simulink model "MATE_HDLsolver_my4thCircuit"  (R2024b)
settings: Solver=FixedStepDiscrete  StartTime=0.0  StopTime=0.05  FixedStep=Ts  MaxStep=100e-6  RelTol=1e-4
PostLoadFcn:
  | Ts=1e-6; nb_sw=3; nb_lc=2;nb_r=1;nb_src=1; nb_out=3; rL=1.2;rC=100;L=1e-3; C=1e-5; Cx=C;LpejoSw=1e-6;h=Ts; MAX_INPUTS=16;
  | MAX_OUTPUTS=16;
  | MAX_SWITCHES=8;
  | MAX_INPUTS=16;
InitFcn:
  | Ts=1e-6; nb_sw=3; nb_lc=2;nb_r=1;nb_src=1; nb_out=3; rL=1.2;rC=100;L=1e-3; C=1e-5; Cx=C;LpejoSw=1e-6;h=Ts; MAX_INPUTS=16;
  | MAX_OUTPUTS=16;
  | MAX_SWITCHES=8;
  | MAX_INPUTS=16;
undefined symbols (not defined in the file or in its folder): MATE_SOC
libraries: fl_lib x35, nesl_utility x13, simetranss x6, ee_lib x4, simulink x3, hdlsllib x3, eeGeneralControl x1
Description:
  | Copyright 2008-2010 The MathWorks, Inc.
settings Model: ARTEMISmethode_block_infos=$$__separator__$$  ModifiedByFormat=Kyle  Creator=Kyle Diller  LastModifiedBy=Kyle
settings SolverCC: AlgebraicLoopSolver=TrustRegion
settings DataIOCC: SaveFormat=Array  SignalLoggingSaveFormat=ModelDataLogs  ReturnWorkspaceOutputs=off  SignalLoggingName=sigsOut
settings OptimizationCC: BlockReduction=off  ConditionallyExecuteInputs=off  OptimizeBlockIOStorage=off  BufferReuse=off  GlobalBufferReuse=off  ExpressionFolding=off  ExpressionDepthLimit=2147483647  LocalBlockOutputs=off  InitFltsAndDblsToZero=on  LifeSpan=inf
settings DebuggingCC: SaveWithParameterizedLinksMsg=none  UnderspecifiedInitializationDetection=Classic  MergeDetectMultiDrivingBlocksExec=none  CheckExecutionContextPreStartOutputMsg=on  SignalResolutionControl=TryResolveAllWithWarning  MultiTaskDSMMsg=warning  MultiTaskCondExecSysMsg=none  SingleTaskRateTransMsg=error  SigSpecEnsureSampleTimeMsg=none  FcnCallInpInsideContextMsg=warning  UnconnectedInputMsg=warning  UnconnectedOutputMsg=warning  UnconnectedLineMsg=warning  AllowSymbolicDim=off  StateNameClashWarn=warning  SFUnexpectedBacktrackingDiag=warning  SFNoUnconditionalDefaultTransitionDiag=warning  SFExecutionAtInitializationDiag=none  ArithmeticOperatorsInVariantConditions=warning
settings HardwareCC: ProdBitPerPointer=32  ProdBitPerSizeT=32  ProdBitPerPtrDiffT=32  ProdLargestAtomicFloat=None  ProdIntDivRoundTo=Undefined  ProdEndianess=Unspecified  ProdWordSize=32  ProdHWDeviceType=Specified  TargetUnknown=on
settings ModelReferenceCC: EnableRefExpFcnMdlSchedulingChecks=on  PropagateSignalLabelsOutOfModel=off
settings SFSimCC: SimUseLocalCustomCode=off  CustomCodeUndefinedFunction=UseInterfaceOnly
settings RTWCC: RTWUseLocalCustomCode=off  GPUComputeCapability=3.5
settings CodeAppCC: StateflowObjectComments=on
settings GRTTargetCC: TargetFcnLib=ansi_tfl_tmw.mat  TargetLangStandard=C89/C90 (ANSI)  CombineOutputUpdateFcns=off  GRTInterface=on
settings ConfigComp: CovMetricSettings=dw  CovSaveCumulativeToWorkspaceVar=on  CovSaveSingleToWorkspaceVar=on  CovExternalEMLEnable=off
settings SimscapeCC: SimscapeNormalizeSystem=off

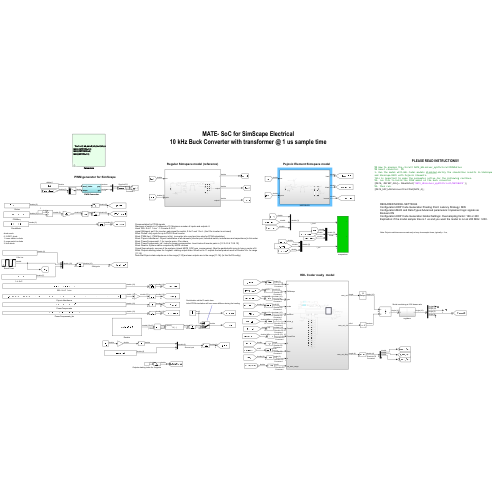
[thumbnail: Simulink's stored preview of the top-level diagram]
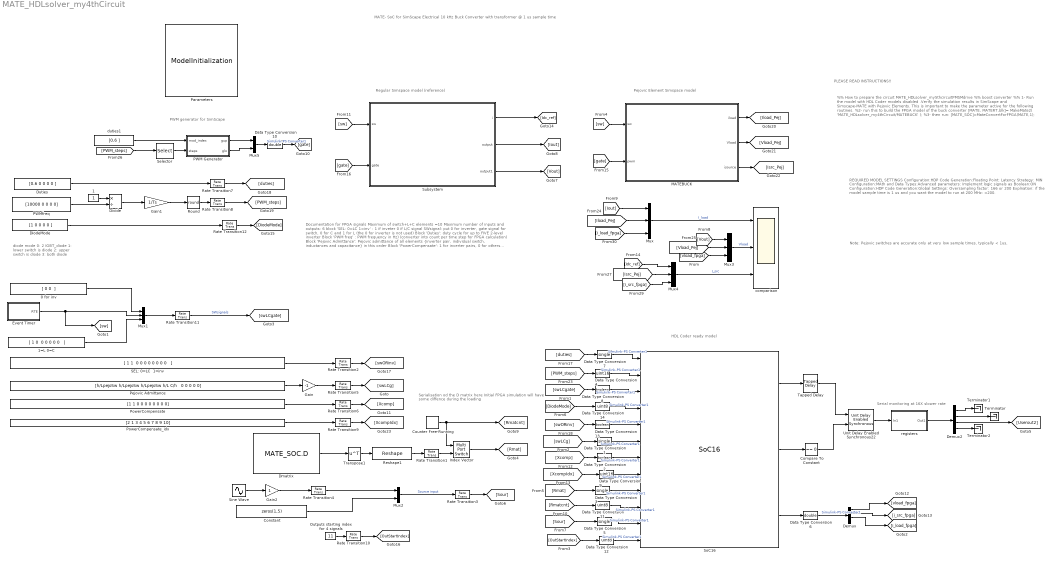
== system MATE_HDLsolver_my4thCircuit ==
  note: Documentation for FPGA signals
      | Maximum of switch+L+C elements =10 Maximum number of inputs and outputs: 6
      | block 'SEL: 0=LC 1=inv' : 1 if inveter 0 if L/C
      | signal SWsignal: put 0 for inverter, gate signal for switch, 0 for C and 1 for L (the 0 for inverter is not used)
      | Block 'Duties': duty cycle for up to FIVE 2-level inverter
      | Block 'PWM freq' : PWM frequency in Hz) (converter into count per time step for FPGA calculation)
      | Block 'Pejovic Admittance': Pejovic admittance of all elements {inverter pair, individual switch, inductances and capacitance} in this order
      | Block 'PowerCompensate': 1 for inverter pairs, 0 for others
      | Block 'PowerCompensate_idx': index for power compensation. Invert index of inverter pairs in [1 2 3 4 5 6 7 8 9 10]
      | Block Dmatrix: System matrix computed by MATE routines
      | Signal SourceInputs: sources of the systems (check MATE_SOC.new_sourcenames). Must be padded with zeros to have a vector of 6
      | Block 'Outputs starting index for 4 signals': starting output index. When set to 11 outputs the last product result of Dmatrix*Vin. for range [11:14]
      | Note that Pejovic state outputs are in the range [1:10] and user outputs are in the range [11:16]. (In this SoCS config)
  note: Serial monitoring at 16X slower rate
  note: Serialisation od the D matrix here
      | Initial FPGA simulation will have some diffence during the loading
  note: Regular Simspace model (reference)
  note: Note: Pejovic switches are accurate only at very low sample times, typically < 1us,
  note: Pejovic Element Simspace model
  note: PLEASE READ INSTRUCTIONS!!
  note: %% How to prepare the circuit MATE_HDLsolver_my5thcircuitPMSMdrive
      | %% boost converter %%
      | 1- Run the model with HDL Coder models disabled .Verify the simulation results in SimScape and Simscape-MATE with Pejovic Elements.
      | This is important to make the parameter active for the following routines.
      | %2- run this to build the FPGA model of the buck converter
      | [MATE, MATERT,blk]= MakeMate2( 'MATE_HDLsolver_my4thCircuit/MATEBUCK' );
      | %3- then run:
      | [MATE_SOC]=MateConvertForFPGA(MATE,1);
  note: HDL Coder ready model
  note: MATE- SoC for SimScape Electrical
      | 10 kHz Buck Converter with transformer @ 1 us sample time
  note: PWM generator for SimScape
  note: diode mode
      | 0: 2 IGBT_diode
      | 1: lower switch is diode
      | 2: upper switch is diode
      | 3: both diode
  note: REQUIRED MODEL SETTINGS
      | Configuration:HDP Code Generation:Floating Point: Latency Strategy: MIN
      | Configuration:MAth and Data Types:Advanced parameters: Implement logic signals as Boolean:ON
      | Configuration:HDP Code Generation:Global Settings: Oversampling factor: 166 or 200
      | Explnation: if the model sample time is 1 us and you want the model to run at 200 MHz: =200.
  " Event Timer" : Subsystem  Tag=RTEcontrol_s38shd7k88  LoadFcn=|  mask(Timer){is=0 (off), t=[0.01 0.02 0.03 0.04 ], Tmax=0.07, Ts=Ts}
      | xx=get_param(gcb,'linkstatus');      
      | if isequal(xx,'inactive')            
      | set_param(gcb,'linkstatus','restore')
      | end
      mask prompts: is "Initial state"; t "Transition times (s):"; Tmax "Repeat period (s)"; Ts "Sample time (s)"
      mask help: This block generates a Simulink control signal changing at specified transition times.
      mask init:
      | iss=get_param(gcb,'is');
      | if isequal(iss,'0 (off)')
      |     sw(1)=0;
      |     sw(2)=0;
      | else
      |     sw(1)=1;
      |     sw(2)=1;
      | end
      | st(1)=0;
      | st(2)=t(1);
      | 
      | if t(1)==0,
      |    h=errordlg(' The first time specified must be greater than 0 ' , 'Parameter error');
      | end
      | 
      | i=3;
      | tog=0;
      | ptr=2;
      | while length(sw)<=2*length(t)
      |     if tog==0
      |         st=[st st(end)+Ts];
      |         sw=[sw 1-sw(end)];
      |         tog=1;
      |     else
      |         st=[st t(ptr)];
      |         sw=[sw sw(end)];
      |         ptr=ptr+1;
      |         tog=0;
      |     end
      | 
      | end
      |  %st=[st Tmax-Ts Tmax+Ts]
      | % sw=[sw sw(end) sw(1)]
      mask TypeOptions is: 0 (off) | 1 (on)
      mask Display:
      | %plot(0,0,100,100,[70,40,40,20,20,13],[30,30,70,70,30,30]);
      | plot( st(1:end-1), sw(1:end-1) );
  0 for inv : Constant  Value="[ 0 0  ]"
  1 : Constant
  1=L 0=C : Constant  Value="[ 1 0  0 0 0 0 0   ]"
  Compare To Constant : hdlsllib/Logic and Bit Operations/Compare To Constant  relop===  const=0  OutDataTypeStr=boolean
  Constant : Constant  Value=zeros(1,5)
  Counter Free-Running : hdlsllib/Sources/Counter Free-Running  NumBits=8  tsamp=-1
  Data Type Conversion{1,3,5,7} (4 alike) : DataTypeConversion  OutDataTypeStr=single  RndMeth=Nearest  SaturateOnIntegerOverflow=off
  Data Type Conversion10 : DataTypeConversion  OutDataTypeStr=double  RndMeth=Nearest  SaturateOnIntegerOverflow=off
  Data Type Conversion11 : DataTypeConversion  OutDataTypeStr=uint8  RndMeth=Nearest  SaturateOnIntegerOverflow=off
  Data Type Conversion12 : DataTypeConversion  OutDataTypeStr=uint8  RndMeth=Nearest  SaturateOnIntegerOverflow=off
  Data Type Conversion13 : DataTypeConversion  OutDataTypeStr=boolean  RndMeth=Nearest  SaturateOnIntegerOverflow=off
  Data Type Conversion14 : DataTypeConversion  OutDataTypeStr=uint8  RndMeth=Nearest  SaturateOnIntegerOverflow=off
  Data Type Conversion2 : DataTypeConversion  OutDataTypeStr=boolean  RndMeth=Nearest  SaturateOnIntegerOverflow=off
  Data Type Conversion4 : DataTypeConversion  OutDataTypeStr=uint16  RndMeth=Nearest  SaturateOnIntegerOverflow=off
  Data Type Conversion6 : DataTypeConversion  OutDataTypeStr=double  RndMeth=Nearest  SaturateOnIntegerOverflow=off
  Data Type Conversion8 : DataTypeConversion  OutDataTypeStr=boolean  RndMeth=Nearest  SaturateOnIntegerOverflow=off
  Data Type Conversion9 : DataTypeConversion  OutDataTypeStr=uint16  RndMeth=Nearest  SaturateOnIntegerOverflow=off
  Demux : Demux
  Demux2 : Demux  Outputs=[nb_sw nb_lc nb_out MAX_OUTPUTS-nb_out-nb_sw-nb_lc]
  DiodeMode : Constant  Value=[1 0 0 0 0 ]
  Divide : Product  Inputs=*/
  Dmatrix : Constant  Value=MATE_SOC.D
  Duties : Constant  Value=[0.6 0 0 0 0 ]
  Gain : Gain  Gain=-1
  Gain1 : Gain  Gain=1/Ts
  Gain2 : Gain
  Index Vector : MultiPortSwitch  DataPortOrder=Zero-based contiguous  Inputs=1  zeroidx=on  SaturateOnIntegerOverflow=off  InputSameDT=off
  MATEBUCK : Subsystem
  Mux{,1,3..4} (4 alike) : Mux  Inputs=3
  Mux2 : Mux  Inputs=2
  Mux5 : Mux  Inputs=2
  Outputs starting index for 4 signals : Constant  Value=11
  PWM Generator : Subsystem  Tag=RTEcontrol_s38shd7k88
  PWMfreq : Constant  Value=[10000 0 0 0 0]
  Parameters : simetranss/Usefulls/ModelInitialization  InitFcnX=|  prel=off  posl=on  inif=on  strf=off
      | Ts=1e-6; nb_sw=3; nb_lc=2;nb_r=1;nb_src=1; nb_out=3; rL=1.2;rC=100;L=1e-3; C=1e-5; Cx=C;LpejoSw=1e-6;h=Ts; MAX_INPUTS=16;
      | MAX_OUTPUTS=16;
      | MAX_SWITCHES=8;
      | MAX_INPUTS=16;
  Pejovic Admittance : Constant  Value="[h/LpejoSw h/LpejoSw h/LpejoSw h/L C/h   0 0 0 0 0]"
  PowerCompensate : Constant  Value=[1 1 0 0 0 0 0 0 0 0]
  PowerCompensate_idx : Constant  Value=[2 1 3 4 5 6 7 8 9 10]
  Rate Transition{1..12} (12 alike) : RateTransition  OutPortSampleTime=1e-06
  Reshape1 : Reshape
  Round : Rounding  Operator=round
  SEL: 0=LC  1=inv : Constant  Value="[ 1 1  0 0 0 0 0 0 0 0   ]"
  Selector : Selector  InputPortWidth=5  IndexOptions=Index vector (dialog)  Indices=1  OutputSizes=1
  Sine Wave : Sin  Amplitude=0  Bias=100  Frequency=0  SampleTime=0
  SoC16 : simetranss/SoC/SoC16  SystemSampleTime=-1  VariantActivationTime=update diagram  AllowFlexibleInterface=on  Latency=0  AutoFrameSizeCalculation=off
  Subsystem : Subsystem
  Tapped Delay : simulink/Discrete/Tapped Delay  vinit=0.0  samptime=-1  NumDelays=16  DelayOrder=Oldest  includeCurrent=off
      settings: LibrarySourceBlock=hdlsllib/Discrete/Tapped Delay
  Terminator : Terminator
  Terminator1 : Terminator
  Terminator2 : Terminator
  Transpose1 : Math  Operator=transpose
  Unit Delay Enabled Synchronous22 : hdlsllib/Discrete/Unit Delay Enabled Synchronous  InitialCondition=0.0  SampleTime=-1
  comparison : Scope  NumInputPorts=3
  duties1 : Constant  Value=[0.6 ]
  registers : Subsystem
  wires:
  Mux/1 -> comparison/1  "I_load"
  Dmatrix/1 -> Transpose1/1
  Sine Wave/1 -> Gain2/1
  Mux3/1 -> comparison/2  "Vload"
  [Vout] -> Mux3/1
  [sw] -> MATEBUCK/1(sw)
  Mux1/1 -> Rate Transition11/1
  Pejovic Admittance/1 -> Gain/1
  Rate Transition5/1 -> [swLCg]
  Gain2/1 -> Rate Transition4/1
  Rate Transition6/1 -> [Xcomp]
  PowerCompensate/1 -> Rate Transition6/1
  [vload_fpga] -> Mux3/3
  [gate] -> MATEBUCK/2(pwm)
  Duties/1 -> Rate Transition7/1
  Rate Transition7/1 -> [duties]
  Mux2/1 -> Rate Transition3/1  "Source input"
  Rate Transition4/1 -> Mux2/1
  Constant/1 -> Mux2/2
  Rate Transition8/1 -> [PWM_steps]
  Divide/1 -> Gain1/1
  Gain1/1 -> Round/1
  Demux2/2 -> Terminator/1
  MATEBUCK/1(iload) -> [Iload_Pej]
  MATEBUCK/2(Vload) -> [Vload_Pej]
  MATEBUCK/3(isource) -> [Isrc_Pej]
  [Iload_Pej] -> Mux/2
  [i_load_fpga] -> Mux/3
  [Vload_Pej] -> Mux3/2
  Mux4/1 -> comparison/3  "I_src"
  [Idc_ref] -> Mux4/1
  [Isrc_Pej] -> Mux4/2
  Demux2/3 -> [Userout2]
  Demux2/1 -> Terminator1/1
  Demux2/4 -> Terminator2/1
  PWMfreq/1 -> Divide/2
  1/1 -> Divide/1
  [i_src_fpga] -> Mux4/3
  PowerCompensate_idx/1 -> Rate Transition9/1
  Rate Transition9/1 -> [XcompIdx]
  Round/1 -> Rate Transition8/1
  duties1/1 -> PWM Generator/1(mod_index)
  [PWM_steps] -> Selector/1
  PWM Generator/2(glo) -> Mux5/2
  PWM Generator/1(gup) -> Mux5/1
  Mux5/1 -> Data Type Conversion10/1
  Data Type Conversion10/1 -> [gate]  "Simulink-PS Converter1"
  [Iout] -> Mux/1
  Transpose1/1 -> Reshape1/1
  Reshape1/1 -> Rate Transition1/1
  Rate Transition1/1 -> Index Vector/2
  Counter Free-Running/1 -> Index Vector/1, [Rmatcnt]
  Index Vector/1 -> [Rmat]
  [Rmatcnt] -> Data Type Conversion11/1
  [swLCg] -> Data Type Conversion1/1
  [XcompIdx] -> Data Type Conversion9/1
  [swLCgate] -> Data Type Conversion8/1
  [Xcomp] -> Data Type Conversion2/1
  [Sour] -> Data Type Conversion5/1
  [Rmat] -> Data Type Conversion3/1
  [duties] -> Data Type Conversion7/1
  Data Type Conversion8/1 -> SoC16/3  "Simulink-PS Converter1"
  Data Type Conversion2/1 -> SoC16/7  "Simulink-PS Converter1"
  Data Type Conversion5/1 -> SoC16/11  "Simulink-PS Converter1"
  Data Type Conversion3/1 -> SoC16/9  "Simulink-PS Converter1"
  [PWM_steps] -> Data Type Conversion4/1
  Data Type Conversion1/1 -> SoC16/6  "Simulink-PS Converter1"
  Data Type Conversion9/1 -> SoC16/8  "Simulink-PS Converter1"
  Data Type Conversion4/1 -> SoC16/2  "Simulink-PS Converter1"
  Data Type Conversion11/1 -> SoC16/10  "Simulink-PS Converter1"
  Data Type Conversion7/1 -> SoC16/1  "Simulink-PS Converter1"
  [gate] -> Subsystem/2(gate)
  Subsystem/1(i) -> [Idc_ref]
  Subsystem/2(output) -> [Iout]
  Subsystem/3(output1) -> [Vout]
  Tapped Delay/1 -> Unit Delay Enabled Synchronous22/1
  SoC16/2 -> Compare To Constant/1
  SoC16/1 -> Tapped Delay/1
  Compare To Constant/1 -> Unit Delay Enabled Synchronous22/2
  Unit Delay Enabled Synchronous22/1 -> registers/1(In1)
  registers/1(Out1) -> Demux2/1
  [OutStartIndex] -> Data Type Conversion12/1
  Data Type Conversion12/1 -> SoC16/12  "Simulink-PS Converter1"
  Rate Transition10/1 -> [OutStartIndex]
  Outputs starting index for 4 signals/1 -> Rate Transition10/1
  [sw] -> Subsystem/1(sw)
  0 for inv/1 -> Mux1/1
  " Event Timer"/1(RTE) -> Mux1/2, [sw]
  Rate Transition11/1 -> [swLCgate]  "SWsignals"
  1=L 0=C/1 -> Mux1/3
  Rate Transition2/1 -> [swORinv]
  SEL: 0=LC  1=inv/1 -> Rate Transition2/1
  [swORinv] -> Data Type Conversion13/1
  Data Type Conversion13/1 -> SoC16/5  "Simulink-PS Converter1"
  Rate Transition3/1 -> [Sour]
  Selector/1 -> PWM Generator/2(steps)
  Gain/1 -> Rate Transition5/1
  Demux/3 -> [i_load_fpga]
  Data Type Conversion6/1 -> Demux/1  "Simulink-PS Converter1"
  Demux/1 -> [vload_fpga]
  Demux/2 -> [i_src_fpga]
  SoC16/3 -> Data Type Conversion6/1
  Rate Transition12/1 -> [DiodeMode]
  DiodeMode/1 -> Rate Transition12/1
  [DiodeMode] -> Data Type Conversion14/1
  Data Type Conversion14/1 -> SoC16/4  "Simulink-PS Converter1"

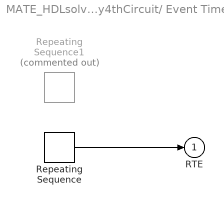
== system MATE_HDLsolver_my4thCircuit/ Event Timer ==
  Repeating Sequence : simulink/Sources/Repeating Sequence  rep_seq_t=st  rep_seq_y=sw
  Repeating Sequence1 : simulink/Sources/Repeating Sequence  Commented=on  rep_seq_t="[0    0.2000    0.2001    0.4000    0.4001    0.6000    2.0000]"  rep_seq_y=|
      | [     1     1     0     0     1     1     1
      | ]
  RTE : Outport  VectorParamsAs1DForOutWhenUnconnected=off
  wires:
  Repeating Sequence/1 -> RTE/1

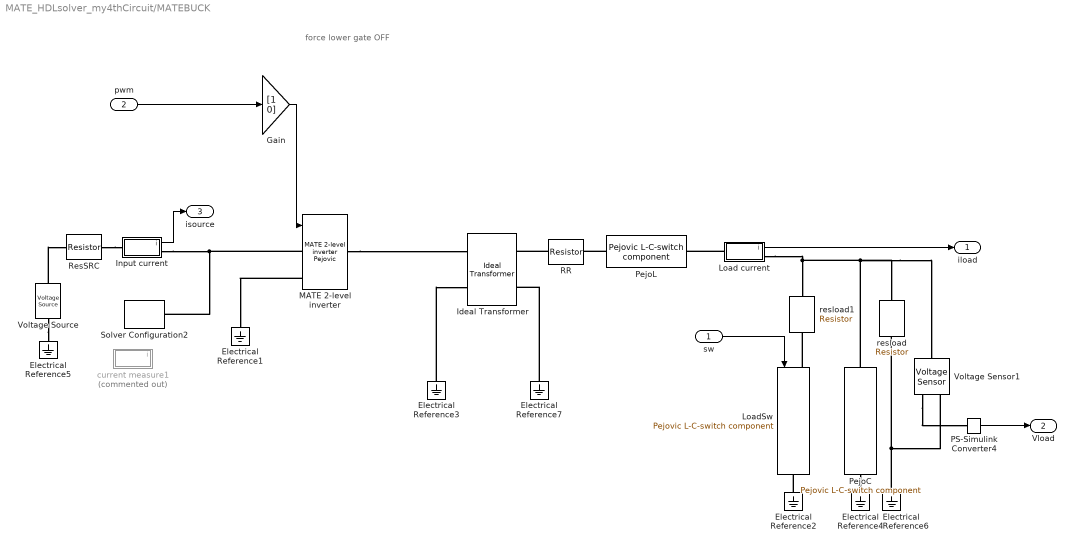
== system MATE_HDLsolver_my4thCircuit/MATEBUCK ==
  note: force lower gate OFF
  sw : Inport
  pwm : Inport  Port=2
  Electrical Reference{1..7} (7 alike) : fl_lib/Electrical/Electrical Elements/Electrical Reference
  Gain : Gain  Gain=[1 0]
  Ideal Transformer : fl_lib/Electrical/Electrical Elements/Ideal Transformer  n=2  i1_specify=off  i1_priority=None  i1=0 A  i1_nominal_specify=off  i1_nominal_value=1  i1_nominal_unit=A  v1_specify=off  v1_priority=None  v1=0 V  v1_nominal_specify=off  v1_nominal_value=1  v1_nominal_unit=V  i2_specify=off  i2_priority=None  i2=0 A  i2_nominal_specify=off  i2_nominal_value=1  i2_nominal_unit=A  v2_specify=off  v2_priority=None  v2=0 V  v2_nominal_specify=off  v2_nominal_value=1  v2_nominal_unit=V
  Input current : Subsystem
  Load current : Subsystem
  LoadSw : simetranss/FPGA/Pejovic L-C-switch component  typ=Switch  Lon=LpejoSw  L=L  C=Cx  traprule=off  otherSW='coming soon'  Ts=Ts  pcbp=off  showV=off  showI=off
  MATE 2-level inverter : simetranss/FPGA/MATE 2-level inverter Pejovic  Lon=1e-6  Ts=Ts
  PS-Simulink Converter4 : nesl_utility/PS-Simulink Converter  PhysicalDomain=network_engine_domain  SubClassName=ps_output  LeftPortType=input  RightPortType=output  PseudoPeriodic=off  Frequencies=[]  VectorFormat=inherit  Unit=inherit  AffineConversion=off
  PejoC : simetranss/FPGA/Pejovic L-C-switch component  typ=Capacitor  Lon=LpejoSw  L=L  C=Cx  traprule=off  otherSW='coming soon'  Ts=Ts  pcbp=off  showV=off  showI=off
  PejoL : simetranss/FPGA/Pejovic L-C-switch component  typ=Inductor  Lon=LpejoSw  L=L  C=C  traprule=off  otherSW='coming soon'  Ts=Ts  pcbp=off  showV=off  showI=off
  RR : fl_lib/Electrical/Electrical Elements/Resistor  R=rL Ohm  i_specify=off  i_priority=None  i=0 A  i_nominal_specify=off  i_nominal_value=1  i_nominal_unit=A  v_specify=off  v_priority=None  v=0 V  v_nominal_specify=off  v_nominal_value=1  v_nominal_unit=V
  ResSRC : fl_lib/Electrical/Electrical Elements/Resistor  R=0.01 Ohm  i_specify=off  i_priority=None  i=0 A  i_nominal_specify=off  i_nominal_value=1  i_nominal_unit=A  v_specify=off  v_priority=None  v=0 V  v_nominal_specify=off  v_nominal_value=1  v_nominal_unit=V
  Solver Configuration2 : nesl_utility/Solver Configuration  PhysicalDomain=network_engine_domain  SubClassName=solver  LeftPortType=input  RightPortType=generic  Tones=[]  Harmonics=[]  SimulateNoise=off  Profile=off  UseLocalSampling=off  EnableSwitchedLinearOptims=on  FrequencyDomain=off  UseCCode=off  RelTol=0.001  AbsTol=0.001  MinStep=1e-09  ToWorkspace=off  RevertToSquareIcSolve=off  NumHomotopyIterations=100  PhasorMode=off  PhasorModeNumHarmonics=1  ConsistencySolver=NEWTON_XTOL_AFTER_FTOL  IndexReductionMethod=DerivativeReplacement  DoDC=off  ResidualTolerance=1e-09  ConsistencyTolSource=GLOBAL  ConsistencyAbsTol=0.001  ConsistencyRelTol=0.001  ConsistencyTolFactor=0.001  UseLocalSolver=on  LocalSolverChoice=NE_BACKWARD_EULER_ADVANCER  ResolveIndetEquations=on  FunctionEvalNumThread=1  LocalSolverSampleTime=Ts  DoFixedCost=on  MaxNonlinIter=1  MaxModeIter=2  ComputeImpulses=off  ImpulseIterations=2  LinearAlgebra=auto  LinearAlgebraNumThread=0  EquationFormulation=NE_TIME_EF  DelaysMemoryBudget=1024  AutomaticFiltering=on  FilteringTimeConstant=0.001  PartitionStorageMethod=AS_NEEDED  PartitionMemoryBudget=1024  PartitionMethod=ROBUST  MultibodyUseLocalSolver=off  MultibodyLocalSolverChoice=ODE1  MultibodyLocalSolverSampleTime=0.001
  Voltage Sensor1 : fl_lib/Electrical/Electrical Sensors/Voltage Sensor
  Voltage Source : ee_lib/Sources/Voltage Source  dc_voltage=100 V  ac_voltage=0 V  ac_shift=0 rad  ac_frequency=60 Hz  noise_mode=ee.enum.sources.noise.Disabled  PSD=0 V^2/Hz  sample_time=1e-3 s  repeatability=ee.enum.sources.repeatability.NotRepeatable  user_seed=0  auto_seed=198304613  i_specify=off  i_priority=None  i=0 A  i_nominal_specify=off  i_nominal_value=1  i_nominal_unit=A  v_specify=off  v_priority=None  v=0 V  v_nominal_specify=off  v_nominal_value=1  v_nominal_unit=V
  current measure1 : Subsystem  Commented=on
      mask Display: disp('amp')
  resload : fl_lib/Electrical/Electrical Elements/Resistor  R=rC Ohm  i_specify=off  i_priority=None  i=0 A  i_nominal_specify=off  i_nominal_value=1  i_nominal_unit=A  v_specify=off  v_priority=None  v=0 V  v_nominal_specify=off  v_nominal_value=1  v_nominal_unit=V
  resload1 : fl_lib/Electrical/Electrical Elements/Resistor  R=rC Ohm  i_specify=off  i_priority=None  i=0 A  i_nominal_specify=off  i_nominal_value=1  i_nominal_unit=A  v_specify=off  v_priority=None  v=0 V  v_nominal_specify=off  v_nominal_value=1  v_nominal_unit=V
  iload : Outport
  Vload : Outport  Port=2
  isource : Outport  Port=3
  wires:
  PS-Simulink Converter4/1 -> Vload/1
  sw/1 -> LoadSw/1
  Load current/1(i) -> iload/1
  pwm/1 -> Gain/1
  Input current/1(i) -> isource/1
  Gain/1 -> MATE 2-level inverter/1
  connections:
  Load current/LConn1 -- PejoL/RConn1
  Voltage Source/RConn1 -- Electrical Reference5/LConn1
  Voltage Source/LConn1 -- ResSRC/LConn1
  PejoL/LConn1 -- RR/RConn1
  PejoC/RConn1 -- Electrical Reference4/LConn1
  Voltage Sensor1/RConn1 -- PS-Simulink Converter4/LConn1
  Electrical Reference6/LConn1 -- resload/RConn1 -- Voltage Sensor1/RConn2
  Input current/RConn1 -- MATE 2-level inverter/LConn1 -- Solver Configuration2/RConn1
  Voltage Sensor1/LConn1 -- resload/LConn1 -- Load current/RConn1 -- resload1/LConn1 -- PejoC/LConn1
  MATE 2-level inverter/LConn2 -- Electrical Reference1/LConn1
  LoadSw/LConn1 -- resload1/RConn1
  Electrical Reference2/LConn1 -- LoadSw/RConn1
  ResSRC/RConn1 -- Input current/LConn1
  RR/LConn1 -- Ideal Transformer/RConn1
  Electrical Reference3/LConn1 -- Ideal Transformer/LConn2
  Electrical Reference7/LConn1 -- Ideal Transformer/RConn2
  MATE 2-level inverter/RConn1 -- Ideal Transformer/LConn1

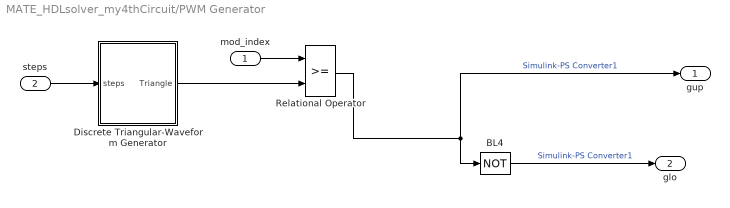
== system MATE_HDLsolver_my4thCircuit/PWM Generator ==
  mod_index : Inport
  steps : Inport  Port=2
  BL4 : Logic  Operator=NOT  Inputs=1
  Discrete Triangular-Waveform Generator : Subsystem
  Relational Operator : RelationalOperator  OutDataTypeStr=boolean
  gup : Outport  VectorParamsAs1DForOutWhenUnconnected=off
  glo : Outport  Port=2  VectorParamsAs1DForOutWhenUnconnected=off
  wires:
  Discrete Triangular-Waveform Generator/1(Triangle) -> Relational Operator/2
  mod_index/1 -> Relational Operator/1
  steps/1 -> Discrete Triangular-Waveform Generator/1(steps)
  Relational Operator/1 -> gup/1, BL4/1  "Simulink-PS Converter1"
  BL4/1 -> glo/1  "Simulink-PS Converter1"

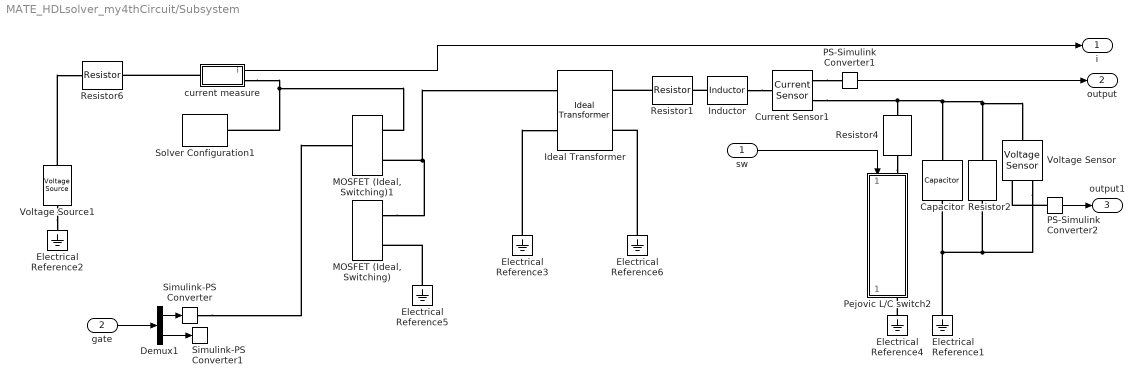
== system MATE_HDLsolver_my4thCircuit/Subsystem ==
  sw : Inport
  gate : Inport  Port=2
  Capacitor : fl_lib/Electrical/Electrical Elements/Capacitor  c=C F  r=0 Ohm  g=0 1/Ohm  i_specify=off  i_priority=None  i=0 A  i_nominal_specify=off  i_nominal_value=1  i_nominal_unit=A  v_specify=off  v_priority=None  v=0 V  v_nominal_specify=off  v_nominal_value=1  v_nominal_unit=V  vc_specify=off  vc_priority=High  vc=0 V  vc_nominal_specify=off  vc_nominal_value=1  vc_nominal_unit=V
  Current Sensor1 : fl_lib/Electrical/Electrical Sensors/Current Sensor
  Demux1 : Demux  Outputs=2
  Electrical Reference{1..6} (6 alike) : fl_lib/Electrical/Electrical Elements/Electrical Reference
  Ideal Transformer : fl_lib/Electrical/Electrical Elements/Ideal Transformer  n=2  i1_specify=off  i1_priority=None  i1=0 A  i1_nominal_specify=off  i1_nominal_value=1  i1_nominal_unit=A  v1_specify=off  v1_priority=None  v1=0 V  v1_nominal_specify=off  v1_nominal_value=1  v1_nominal_unit=V  i2_specify=off  i2_priority=None  i2=0 A  i2_nominal_specify=off  i2_nominal_value=1  i2_nominal_unit=A  v2_specify=off  v2_priority=None  v2=0 V  v2_nominal_specify=off  v2_nominal_value=1  v2_nominal_unit=V
  Inductor : fl_lib/Electrical/Electrical Elements/Inductor  l=L H  r=0 Ohm  g=1e-9 1/Ohm  i_specify=off  i_priority=None  i=0 A  i_nominal_specify=off  i_nominal_value=1  i_nominal_unit=A  v_specify=off  v_priority=None  v=0 V  v_nominal_specify=off  v_nominal_value=1  v_nominal_unit=V  i_L_specify=off  i_L_priority=High  i_L=0 A  i_L_nominal_specify=off  i_L_nominal_value=1  i_L_nominal_unit=A
  "MOSFET (Ideal, Switching)" : ee_lib/Semiconductors & Converters/MOSFET (Ideal, Switching)  port_option=ee.enum.controlport.ps  Rds=0.001 Ohm  Goff=1e-6 1/Ohm  Vth=0.1 V  diode_param=ee.enum.semiconductors.protectionDiode.nodynamics  diode_Vf=0.001 V  diode_Ron=0.001 Ohm  diode_Goff=1e-6 1/Ohm  diode_C=50e-9 F  diode_iRM=-235 A  diode_iF=300 A  diode_idot=-50 A/us  diode_trr_param=ee.enum.converters.diodeReverseParam.trr_factor  diode_trr_factor=3  diode_trr=15 us  diode_Qrr=1500 s*uA  ids_specify=off  ids_priority=None  ids=0 A  ids_nominal_specify=off  ids_nominal_value=1  ids_nominal_unit=A  vds_specify=off  vds_priority=None  vds=0 V  vds_nominal_specify=off  vds_nominal_value=1  vds_nominal_unit=V  vgs_specify=off  vgs_priority=None  vgs=0 V  vgs_nominal_specify=off  vgs_nominal_value=1  vgs_nominal_unit=V  thermal_loss_option=ee.enum.converters.thermalLossOption.constantvalues  Von_data=[0, 1.8, 3.2, 6, 10, 16; 0, 2, 5.5, 9.5, 15, 25] V  Tj=[298.15, 448.15] K  Iout_data=[0, 20, 40, 60, 80, 100] A  Eon_data=[0, 55.04, 124.57, 235.53, 362.12; 0, 71.25, 161.25, 304.88, 468.75] * 1e-6 J  Eoff_data=[0, 18, 30, 56.1, 76.5; 0, 22.5, 37.5, 70.13, 95.63] * 1e-6 J  Eon_data_3D=[zeros(2, 5, 3)] J  Eoff_data_3D=[zeros(2, 5, 3)] J  Tj_loss=[298.15, 448.15] K  Iout_data_loss=[0, 10, 20, 30, 40] A  tabulateWithVds=false  Vds_loss=[0, 150, 300] V  Eon_scalar=22.86e-3 J  Eoff_scalar=17.14e-3 J  Voff=300 V  Iout_scalar=600 A  useCurrentFromPreviousCycle=false  useVoltageFromPreviousCycle=false  diodeModelType=ee.enum.converters.diodeModelType.pwl  diodeTableType=ee.enum.diode.tableType.IfMat  diode_ReverseIVType=ee.enum.diode.diodeReverseIV.constant  diode_IfMat=[.07, .12, .19, 1.75, 4.24, 7.32, 11.2; .16, .3, .72, 2.14, 4.02, 6.35, 9.12] A  diode_VfMat=[.9, 1.15, 1.25, 1.5, 1.75, 2.17, 2.6, 2.85; .58, .68, .75, 1.1, 1.38, 1.77, 2.27, 2.7] V  diode_TjVec=[25, 125] degC  diode_VfVec=[.5, .7, .9, 1.3, 1.7, 2.1, 2.5] V  diode_IfVec=[.1, .2, .5, 1, 2, 4, 7, 10] A  diode_IrMat=[1e-06, 2e-06, 5e-06, 1e-05, 2.5e-05, 5e-05, .0001; 2e-06, 5e-06, 1e-05, 4e-05, 8e-05, .0002, .0005] A  diode_VrMat=[10, 100, 200, 250, 300, 325, 350; 10, 70, 160, 220, 270, 300, 320] V  diode_VrVec=[10, 20, 40, 50, 70, 80, 100] V  diode_IrVec=[1e-06, 2e-06, 5e-06, 1e-05, 2e-05, 5e-05, .0001] A  diode_Vr=-600 V  diode_Ls=150 nH  diode_Erec=0.03 J  diode_rec_loss_model=ee.enum.diode.reverseRecoveryModel.fixed  diode_ErecVal=0 J  diode_scaleWithIandV=true  diode_ErecMat=zeros(2, 3) J  diode_TjrecVec=[298.15, 398.15] K  diode_IfrecVec=[.1, 1, 10] A  diode_IrecVal=10 A  diode_VrecVal=10 V  diode_tFilter=1 / 1000 / 100 s  separateThermalPortForDiode=false  thermal_network_parameterization=ee.enum.thermalNetworkTopology.external  Rth=[.03, .2] K/W  Rth_Cauer=[.03, .1, .2] K/W  Rth_Foster=[.08, .14, .22, .16] K/W  thermal_mass_parameterization=ee.enum.thermalNetwork.timeconstant  thermal_mass=[3, 25] J/K  thermal_mass_Cauer=[3, 10, 25] J/K  thermal_mass_Foster=[.001, .005, .05, .5] J/K  thermal_time_constant=[.1, 5] s  thermal_time_constant_Cauer=[.1, 1, 5] s  thermal_time_constant_Foster=[7e-05, .0007, .01, .08] s  thermal_mass_initial_temperatures=[25, 25] degC  thermal_mass_initial_temperatures_Cauer=[25, 25, 25] degC  junction_thermal_mass=0.1 J/K  Tvec_initial_Foster=[25, 25, 25, 25] degC  RthDiode=[.03, .2] K/W  RthCauerDiode=[.03, .1, .2] K/W  RthFosterDiode=[.03, .2] K/W  thermalMassDiode=[3, 25] J/K  thermalMassCauerDiode=[3, 10, 25] J/K  thermalMassFosterDiode=[33, 50] J/K  thermalTauDiode=[.1, 5] s  thermalTauCauerDiode=[.1, 1, 5] s  thermalTauFosterDiode=[1, 10] s  thermalMassInitTempDiode=[25, 25] degC  thermalMassInitTempCauerDiode=[25, 25, 25] degC  junctionthermalMassDiode=0.1 J/K  TVecInitialFosterDiode=[25, 25, 25, 25] degC  no_thermal_network=0  mosfet_junction_temperature_specify=off  mosfet_junction_temperature_priority=None  mosfet_junction_temperature=25 degC  mosfet_junction_temperature_nominal_specify=off  mosfet_junction_temperature_nominal_value=1  mosfet_junction_temperature_nominal_unit=degC  diode_junction_temperature_specify=off  diode_junction_temperature_priority=None  diode_junction_temperature=25 degC  diode_junction_temperature_nominal_specify=off  diode_junction_temperature_nominal_value=1  diode_junction_temperature_nominal_unit=degC  Qj_specify=off  Qj_priority=None  Qj=0 W  Qj_nominal_specify=off  Qj_nominal_value=1  Qj_nominal_unit=W  accumulatedSwitchingLosses_specify=off  accumulatedSwitchingLosses_priority=None  accumulatedSwitchingLosses=0 J
  "MOSFET (Ideal, Switching)1" : ee_lib/Semiconductors & Converters/MOSFET (Ideal, Switching)  port_option=ee.enum.controlport.ps  Rds=0.001 Ohm  Goff=1e-6 1/Ohm  Vth=0.1 V  diode_param=ee.enum.semiconductors.protectionDiode.nodynamics  diode_Vf=0.001 V  diode_Ron=0.001 Ohm  diode_Goff=1e-6 1/Ohm  diode_C=50e-9 F  diode_iRM=-235 A  diode_iF=300 A  diode_idot=-50 A/us  diode_trr_param=ee.enum.converters.diodeReverseParam.trr_factor  diode_trr_factor=3  diode_trr=15 us  diode_Qrr=1500 s*uA  ids_specify=off  ids_priority=None  ids=0 A  ids_nominal_specify=off  ids_nominal_value=1  ids_nominal_unit=A  vds_specify=off  vds_priority=None  vds=0 V  vds_nominal_specify=off  vds_nominal_value=1  vds_nominal_unit=V  vgs_specify=off  vgs_priority=None  vgs=0 V  vgs_nominal_specify=off  vgs_nominal_value=1  vgs_nominal_unit=V  thermal_loss_option=ee.enum.converters.thermalLossOption.constantvalues  Von_data=[0, 1.8, 3.2, 6, 10, 16; 0, 2, 5.5, 9.5, 15, 25] V  Tj=[298.15, 448.15] K  Iout_data=[0, 20, 40, 60, 80, 100] A  Eon_data=[0, 55.04, 124.57, 235.53, 362.12; 0, 71.25, 161.25, 304.88, 468.75] * 1e-6 J  Eoff_data=[0, 18, 30, 56.1, 76.5; 0, 22.5, 37.5, 70.13, 95.63] * 1e-6 J  Eon_data_3D=[zeros(2, 5, 3)] J  Eoff_data_3D=[zeros(2, 5, 3)] J  Tj_loss=[298.15, 448.15] K  Iout_data_loss=[0, 10, 20, 30, 40] A  tabulateWithVds=false  Vds_loss=[0, 150, 300] V  Eon_scalar=22.86e-3 J  Eoff_scalar=17.14e-3 J  Voff=300 V  Iout_scalar=600 A  useCurrentFromPreviousCycle=false  useVoltageFromPreviousCycle=false  diodeModelType=ee.enum.converters.diodeModelType.pwl  diodeTableType=ee.enum.diode.tableType.IfMat  diode_ReverseIVType=ee.enum.diode.diodeReverseIV.constant  diode_IfMat=[.07, .12, .19, 1.75, 4.24, 7.32, 11.2; .16, .3, .72, 2.14, 4.02, 6.35, 9.12] A  diode_VfMat=[.9, 1.15, 1.25, 1.5, 1.75, 2.17, 2.6, 2.85; .58, .68, .75, 1.1, 1.38, 1.77, 2.27, 2.7] V  diode_TjVec=[25, 125] degC  diode_VfVec=[.5, .7, .9, 1.3, 1.7, 2.1, 2.5] V  diode_IfVec=[.1, .2, .5, 1, 2, 4, 7, 10] A  diode_IrMat=[1e-06, 2e-06, 5e-06, 1e-05, 2.5e-05, 5e-05, .0001; 2e-06, 5e-06, 1e-05, 4e-05, 8e-05, .0002, .0005] A  diode_VrMat=[10, 100, 200, 250, 300, 325, 350; 10, 70, 160, 220, 270, 300, 320] V  diode_VrVec=[10, 20, 40, 50, 70, 80, 100] V  diode_IrVec=[1e-06, 2e-06, 5e-06, 1e-05, 2e-05, 5e-05, .0001] A  diode_Vr=-600 V  diode_Ls=150 nH  diode_Erec=0.03 J  diode_rec_loss_model=ee.enum.diode.reverseRecoveryModel.fixed  diode_ErecVal=0 J  diode_scaleWithIandV=true  diode_ErecMat=zeros(2, 3) J  diode_TjrecVec=[298.15, 398.15] K  diode_IfrecVec=[.1, 1, 10] A  diode_IrecVal=10 A  diode_VrecVal=10 V  diode_tFilter=1 / 1000 / 100 s  separateThermalPortForDiode=false  thermal_network_parameterization=ee.enum.thermalNetworkTopology.external  Rth=[.03, .2] K/W  Rth_Cauer=[.03, .1, .2] K/W  Rth_Foster=[.08, .14, .22, .16] K/W  thermal_mass_parameterization=ee.enum.thermalNetwork.timeconstant  thermal_mass=[3, 25] J/K  thermal_mass_Cauer=[3, 10, 25] J/K  thermal_mass_Foster=[.001, .005, .05, .5] J/K  thermal_time_constant=[.1, 5] s  thermal_time_constant_Cauer=[.1, 1, 5] s  thermal_time_constant_Foster=[7e-05, .0007, .01, .08] s  thermal_mass_initial_temperatures=[25, 25] degC  thermal_mass_initial_temperatures_Cauer=[25, 25, 25] degC  junction_thermal_mass=0.1 J/K  Tvec_initial_Foster=[25, 25, 25, 25] degC  RthDiode=[.03, .2] K/W  RthCauerDiode=[.03, .1, .2] K/W  RthFosterDiode=[.03, .2] K/W  thermalMassDiode=[3, 25] J/K  thermalMassCauerDiode=[3, 10, 25] J/K  thermalMassFosterDiode=[33, 50] J/K  thermalTauDiode=[.1, 5] s  thermalTauCauerDiode=[.1, 1, 5] s  thermalTauFosterDiode=[1, 10] s  thermalMassInitTempDiode=[25, 25] degC  thermalMassInitTempCauerDiode=[25, 25, 25] degC  junctionthermalMassDiode=0.1 J/K  TVecInitialFosterDiode=[25, 25, 25, 25] degC  no_thermal_network=0  mosfet_junction_temperature_specify=off  mosfet_junction_temperature_priority=None  mosfet_junction_temperature=25 degC  mosfet_junction_temperature_nominal_specify=off  mosfet_junction_temperature_nominal_value=1  mosfet_junction_temperature_nominal_unit=degC  diode_junction_temperature_specify=off  diode_junction_temperature_priority=None  diode_junction_temperature=25 degC  diode_junction_temperature_nominal_specify=off  diode_junction_temperature_nominal_value=1  diode_junction_temperature_nominal_unit=degC  Qj_specify=off  Qj_priority=None  Qj=0 W  Qj_nominal_specify=off  Qj_nominal_value=1  Qj_nominal_unit=W  accumulatedSwitchingLosses_specify=off  accumulatedSwitchingLosses_priority=None  accumulatedSwitchingLosses=0 J
  PS-Simulink Converter1 : nesl_utility/PS-Simulink Converter  PhysicalDomain=network_engine_domain  SubClassName=ps_output  LeftPortType=input  RightPortType=output  PseudoPeriodic=off  Frequencies=[]  VectorFormat=inherit  Unit=inherit  AffineConversion=off
  PS-Simulink Converter2 : nesl_utility/PS-Simulink Converter  PhysicalDomain=network_engine_domain  SubClassName=ps_output  LeftPortType=input  RightPortType=output  PseudoPeriodic=off  Frequencies=[]  VectorFormat=inherit  Unit=inherit  AffineConversion=off
  Pejovic L/C switch2 : Subsystem  AncestorBlock=simetranss/FPGA/Pejovic L//C switch  mask(Pejovic Switch){Lon=LpejoSw, Ts=Ts}
      mask prompts: Lon "Selected equivalent ON inductance (H)"; Ts "Sample Time (s)"
      mask help:
      | Pejovic switch model in SimScape
      |
      | Implements a single phase switch model using the Pejovic constant admittance method.
      | The user only has to select the equivalent ON-state inductance of the model, the corresponding Capacitance is computed internally.
      |
      | In the Pejovic model, Ts/Lon=Coff/Ts (Backward Euler) resulting in a constant admittance for the DAE solver.
      |
      | Input signals;
      |
      | gate: the switch gate value (1 for ON , 0 for OFF)
      mask init:
      | Coff=Ts*Ts/Lon;
      | Rsw=Lon/Ts;
      | 
      | if Ts>2e-6
      |     warndlg(['Sample Time of ' num2str(Ts) ' s. may be somehow large for the Pejovic switch to be accurate. Sample time below 2 us are recommended.'])
      | end
      mask Display: disp(['Pswitch'])
  Resistor1 : fl_lib/Electrical/Electrical Elements/Resistor  R=rL Ohm  i_specify=off  i_priority=None  i=0 A  i_nominal_specify=off  i_nominal_value=1  i_nominal_unit=A  v_specify=off  v_priority=None  v=0 V  v_nominal_specify=off  v_nominal_value=1  v_nominal_unit=V
  Resistor2 : fl_lib/Electrical/Electrical Elements/Resistor  R=rC Ohm  i_specify=off  i_priority=None  i=0 A  i_nominal_specify=off  i_nominal_value=1  i_nominal_unit=A  v_specify=off  v_priority=None  v=0 V  v_nominal_specify=off  v_nominal_value=1  v_nominal_unit=V
  Resistor4 : fl_lib/Electrical/Electrical Elements/Resistor  R=rC Ohm  i_specify=off  i_priority=None  i=0 A  i_nominal_specify=off  i_nominal_value=1  i_nominal_unit=A  v_specify=off  v_priority=None  v=0 V  v_nominal_specify=off  v_nominal_value=1  v_nominal_unit=V
  Resistor6 : fl_lib/Electrical/Electrical Elements/Resistor  R=0.01 Ohm  i_specify=off  i_priority=None  i=0 A  i_nominal_specify=off  i_nominal_value=1  i_nominal_unit=A  v_specify=off  v_priority=None  v=0 V  v_nominal_specify=off  v_nominal_value=1  v_nominal_unit=V
  Simulink-PS Converter : nesl_utility/Simulink-PS Converter  PhysicalDomain=network_engine_domain  SubClassName=ps_input  LeftPortType=input  RightPortType=output  PseudoPeriodic=off  Frequencies=[]  NoiseDistribution=none  NoiseParameters=[]  Unit=1  AffineConversion=off  FilteringAndDerivatives=provide  SimscapeFilterOrder=1  InputFilterTimeConstant=0.001  UdotUserProvided=0
  Simulink-PS Converter1 : nesl_utility/Simulink-PS Converter  PhysicalDomain=network_engine_domain  SubClassName=ps_input  LeftPortType=input  RightPortType=output  PseudoPeriodic=off  Frequencies=[]  NoiseDistribution=none  NoiseParameters=[]  Unit=1  AffineConversion=off  FilteringAndDerivatives=provide  SimscapeFilterOrder=1  InputFilterTimeConstant=0.001  UdotUserProvided=0
  Solver Configuration1 : nesl_utility/Solver Configuration  PhysicalDomain=network_engine_domain  SubClassName=solver  LeftPortType=input  RightPortType=generic  Tones=[]  Harmonics=[]  SimulateNoise=off  Profile=off  UseLocalSampling=off  EnableSwitchedLinearOptims=on  FrequencyDomain=off  UseCCode=off  RelTol=0.001  AbsTol=0.001  MinStep=1e-09  ToWorkspace=off  RevertToSquareIcSolve=off  NumHomotopyIterations=100  PhasorMode=off  PhasorModeNumHarmonics=1  ConsistencySolver=NEWTON_XTOL_AFTER_FTOL  IndexReductionMethod=DerivativeReplacement  DoDC=off  ResidualTolerance=1e-09  ConsistencyTolSource=GLOBAL  ConsistencyAbsTol=0.001  ConsistencyRelTol=0.001  ConsistencyTolFactor=0.001  UseLocalSolver=on  LocalSolverChoice=NE_BACKWARD_EULER_ADVANCER  ResolveIndetEquations=on  FunctionEvalNumThread=1  LocalSolverSampleTime=Ts  DoFixedCost=on  MaxNonlinIter=2  MaxModeIter=2  ComputeImpulses=off  ImpulseIterations=2  LinearAlgebra=auto  LinearAlgebraNumThread=0  EquationFormulation=NE_TIME_EF  DelaysMemoryBudget=1024  AutomaticFiltering=on  FilteringTimeConstant=0.001  PartitionStorageMethod=AS_NEEDED  PartitionMemoryBudget=1024  PartitionMethod=ROBUST  MultibodyUseLocalSolver=off  MultibodyLocalSolverChoice=ODE1  MultibodyLocalSolverSampleTime=0.001
  Voltage Sensor : fl_lib/Electrical/Electrical Sensors/Voltage Sensor
  Voltage Source1 : ee_lib/Sources/Voltage Source  dc_voltage=100 V  ac_voltage=0 V  ac_shift=0 rad  ac_frequency=60 Hz  noise_mode=ee.enum.sources.noise.Disabled  PSD=0 V^2/Hz  sample_time=1e-3 s  repeatability=ee.enum.sources.repeatability.NotRepeatable  user_seed=0  auto_seed=1196140742  i_specify=off  i_priority=None  i=0 A  i_nominal_specify=off  i_nominal_value=1  i_nominal_unit=A  v_specify=off  v_priority=None  v=0 V  v_nominal_specify=off  v_nominal_value=1  v_nominal_unit=V
  current measure : Subsystem
      mask Display: disp('amp')
  i : Outport
  output : Outport  Port=2
  output1 : Outport  Port=3
  wires:
  sw/1 -> Pejovic L/C switch2/1(gate)
  Demux1/2 -> Simulink-PS Converter1/1
  current measure/1(i) -> i/1
  Demux1/1 -> Simulink-PS Converter/1
  gate/1 -> Demux1/1
  PS-Simulink Converter1/1 -> output/1
  PS-Simulink Converter2/1 -> output1/1
  connections:
  Electrical Reference4/LConn1 -- Pejovic L/C switch2/RConn1
  current measure/RConn1 -- "MOSFET (Ideal, Switching)1"/RConn1 -- Solver Configuration1/RConn1
  Current Sensor1/RConn2 -- Resistor4/LConn1 -- Voltage Sensor/LConn1 -- Resistor2/LConn1 -- Capacitor/LConn1
  Voltage Sensor/RConn2 -- Resistor2/RConn1 -- Capacitor/RConn1 -- Electrical Reference1/LConn1
  Resistor4/RConn1 -- Pejovic L/C switch2/LConn1
  current measure/LConn1 -- Resistor6/RConn1
  Voltage Source1/LConn1 -- Resistor6/LConn1
  PS-Simulink Converter2/LConn1 -- Voltage Sensor/RConn1
  Inductor/RConn1 -- Current Sensor1/LConn1
  Inductor/LConn1 -- Resistor1/RConn1
  Current Sensor1/RConn1 -- PS-Simulink Converter1/LConn1
  Voltage Source1/RConn1 -- Electrical Reference2/LConn1
  "MOSFET (Ideal, Switching)"/RConn1 -- Ideal Transformer/LConn1 -- "MOSFET (Ideal, Switching)1"/RConn2
  Electrical Reference5/LConn1 -- "MOSFET (Ideal, Switching)"/RConn2
  Simulink-PS Converter/RConn1 -- "MOSFET (Ideal, Switching)1"/LConn1
  Resistor1/LConn1 -- Ideal Transformer/RConn1
  Electrical Reference3/LConn1 -- Ideal Transformer/LConn2
  Electrical Reference6/LConn1 -- Ideal Transformer/RConn2

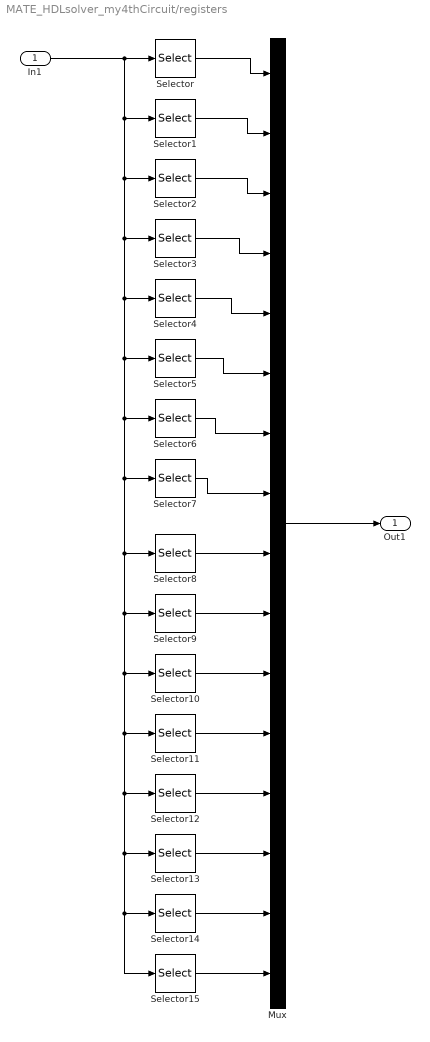
== system MATE_HDLsolver_my4thCircuit/registers ==
  In1 : Inport
  Mux : Mux  Inputs=16
  Selector : Selector  InputPortWidth=16  IndexOptions=Index vector (dialog)  Indices=1  OutputSizes=1
  Selector1 : Selector  InputPortWidth=16  IndexOptions=Index vector (dialog)  Indices=2  OutputSizes=1
  Selector10 : Selector  InputPortWidth=16  IndexOptions=Index vector (dialog)  Indices=11  OutputSizes=1
  Selector11 : Selector  InputPortWidth=16  IndexOptions=Index vector (dialog)  Indices=12  OutputSizes=1
  Selector12 : Selector  InputPortWidth=16  IndexOptions=Index vector (dialog)  Indices=13  OutputSizes=1
  Selector13 : Selector  InputPortWidth=16  IndexOptions=Index vector (dialog)  Indices=14  OutputSizes=1
  Selector14 : Selector  InputPortWidth=16  IndexOptions=Index vector (dialog)  Indices=15  OutputSizes=1
  Selector15 : Selector  InputPortWidth=16  IndexOptions=Index vector (dialog)  Indices=16  OutputSizes=1
  Selector2 : Selector  InputPortWidth=16  IndexOptions=Index vector (dialog)  Indices=3  OutputSizes=1
  Selector3 : Selector  InputPortWidth=16  IndexOptions=Index vector (dialog)  Indices=4  OutputSizes=1
  Selector4 : Selector  InputPortWidth=16  IndexOptions=Index vector (dialog)  Indices=5  OutputSizes=1
  Selector5 : Selector  InputPortWidth=16  IndexOptions=Index vector (dialog)  Indices=6  OutputSizes=1
  Selector6 : Selector  InputPortWidth=16  IndexOptions=Index vector (dialog)  Indices=7  OutputSizes=1
  Selector7 : Selector  InputPortWidth=16  IndexOptions=Index vector (dialog)  Indices=8  OutputSizes=1
  Selector8 : Selector  InputPortWidth=16  IndexOptions=Index vector (dialog)  Indices=9  OutputSizes=1
  Selector9 : Selector  InputPortWidth=16  IndexOptions=Index vector (dialog)  Indices=10  OutputSizes=1
  Out1 : Outport
  wires:
  In1/1 -> Selector/1, Selector1/1, Selector2/1, Selector3/1, Selector4/1, Selector5/1, Selector6/1, Selector7/1, Selector8/1, Selector9/1, Selector10/1, Selector11/1, Selector12/1, Selector13/1, Selector15/1, Selector14/1
  Selector8/1 -> Mux/9
  Selector9/1 -> Mux/10
  Selector10/1 -> Mux/11
  Selector11/1 -> Mux/12
  Selector12/1 -> Mux/13
  Selector13/1 -> Mux/14
  Selector14/1 -> Mux/15
  Selector15/1 -> Mux/16
  Selector/1 -> Mux/1
  Selector1/1 -> Mux/2
  Selector2/1 -> Mux/3
  Selector3/1 -> Mux/4
  Selector4/1 -> Mux/5
  Selector5/1 -> Mux/6
  Selector6/1 -> Mux/7
  Selector7/1 -> Mux/8
  Mux/1 -> Out1/1

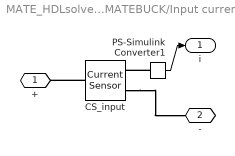
== system MATE_HDLsolver_my4thCircuit/MATEBUCK/Input current ==
  CS_input : fl_lib/Electrical/Electrical Sensors/Current Sensor
  PS-Simulink Converter1 : nesl_utility/PS-Simulink Converter  PhysicalDomain=network_engine_domain  SubClassName=ps_output  LeftPortType=input  RightPortType=output  PseudoPeriodic=off  Frequencies=[]  VectorFormat=inherit  Unit=inherit  AffineConversion=off
  + : PMIOPort  Side=Left
  - : PMIOPort  Port=2  Side=Right
  i : Outport
  wires:
  PS-Simulink Converter1/1 -> i/1
  connections:
  PS-Simulink Converter1/LConn1 -- CS_input/RConn1
  CS_input/LConn1 -- +/RConn1
  CS_input/RConn2 -- -/RConn1

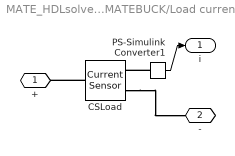
== system MATE_HDLsolver_my4thCircuit/MATEBUCK/Load current ==
  CSLoad : fl_lib/Electrical/Electrical Sensors/Current Sensor
  PS-Simulink Converter1 : nesl_utility/PS-Simulink Converter  PhysicalDomain=network_engine_domain  SubClassName=ps_output  LeftPortType=input  RightPortType=output  PseudoPeriodic=off  Frequencies=[]  VectorFormat=inherit  Unit=inherit  AffineConversion=off
  + : PMIOPort  Side=Left
  - : PMIOPort  Port=2  Side=Right
  i : Outport
  wires:
  PS-Simulink Converter1/1 -> i/1
  connections:
  CSLoad/RConn2 -- -/RConn1
  CSLoad/LConn1 -- +/RConn1
  PS-Simulink Converter1/LConn1 -- CSLoad/RConn1

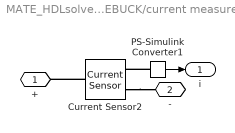
== system MATE_HDLsolver_my4thCircuit/MATEBUCK/current measure1 ==
  Current Sensor2 : fl_lib/Electrical/Electrical Sensors/Current Sensor
  PS-Simulink Converter1 : nesl_utility/PS-Simulink Converter  PhysicalDomain=network_engine_domain  SubClassName=ps_output  LeftPortType=input  RightPortType=output  PseudoPeriodic=off  Frequencies=[]  VectorFormat=inherit  Unit=inherit  AffineConversion=off
  + : PMIOPort  Side=Left
  - : PMIOPort  Port=2  Side=Right
  i : Outport
  wires:
  PS-Simulink Converter1/1 -> i/1
  connections:
  Current Sensor2/RConn2 -- -/RConn1
  Current Sensor2/LConn1 -- +/RConn1
  PS-Simulink Converter1/LConn1 -- Current Sensor2/RConn1

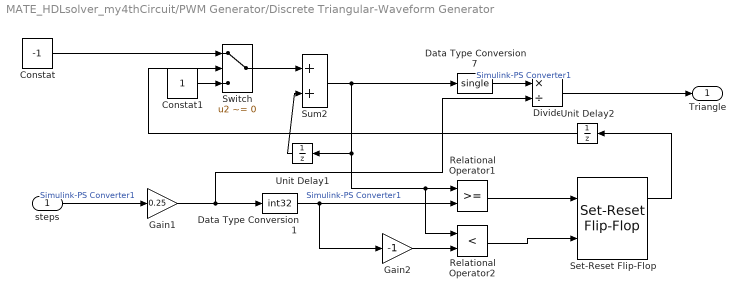
== system MATE_HDLsolver_my4thCircuit/PWM Generator/Discrete Triangular-Waveform Generator ==
  steps : Inport
  Constat : Constant  Value=-1  OutDataTypeStr=int32
  Constat1 : Constant  OutDataTypeStr=int32
  Data Type Conversion1 : DataTypeConversion  OutDataTypeStr=int32  RndMeth=Nearest  SaturateOnIntegerOverflow=off
  Data Type Conversion7 : DataTypeConversion  OutDataTypeStr=single  RndMeth=Nearest  SaturateOnIntegerOverflow=off
  Divide : Product  Inputs=*/
  Gain1 : Gain  Gain=0.25  SaturateOnIntegerOverflow=on  OutDataTypeStr=Inherit: Same as input  ParamDataTypeStr=Inherit: Same as input
  Gain2 : Gain  Gain=-1  SaturateOnIntegerOverflow=on  OutDataTypeStr=Inherit: Same as input  ParamDataTypeStr=Inherit: Same as input
  Relational Operator1 : RelationalOperator
  Relational Operator2 : RelationalOperator  Operator=<
  Set-Reset Flip-Flop : eeGeneralControl/Set-Reset Flip-Flop  LabelModeActiveChoice=Discrete  UndefState=Set  Q0=0  Ts=Ts
      settings: LibrarySourceBlock=ee_sl_lib/General Control/Set-Reset Flip-Flop
  Sum2 : Sum  InputSameDT=on  SaturateOnIntegerOverflow=on  OutDataTypeStr=Inherit: Same as first input
  Switch : Switch  Criteria=u2 ~= 0
  Unit Delay1 : UnitDelay  SampleTime=Ts  HasFrameUpgradeWarning=on
  Unit Delay2 : UnitDelay  SampleTime=Ts  HasFrameUpgradeWarning=on
  Triangle : Outport  InitialOutput=0  VectorParamsAs1DForOutWhenUnconnected=off
  wires:
  Constat/1 -> Switch/1
  Constat1/1 -> Switch/3
  Switch/1 -> Sum2/1
  Unit Delay1/1 -> Sum2/2
  Sum2/1 -> Relational Operator2/1, Relational Operator1/1, Unit Delay1/1, Data Type Conversion7/1
  Gain1/1 -> Divide/2, Data Type Conversion1/1
  Relational Operator1/1 -> Set-Reset Flip-Flop/1
  Gain2/1 -> Relational Operator2/2
  Relational Operator2/1 -> Set-Reset Flip-Flop/2
  Set-Reset Flip-Flop/1 -> Unit Delay2/1
  Unit Delay2/1 -> Switch/2
  Divide/1 -> Triangle/1
  Data Type Conversion7/1 -> Divide/1  "Simulink-PS Converter1"
  steps/1 -> Gain1/1  "Simulink-PS Converter1"
  Data Type Conversion1/1 -> Gain2/1, Relational Operator1/2  "Simulink-PS Converter1"

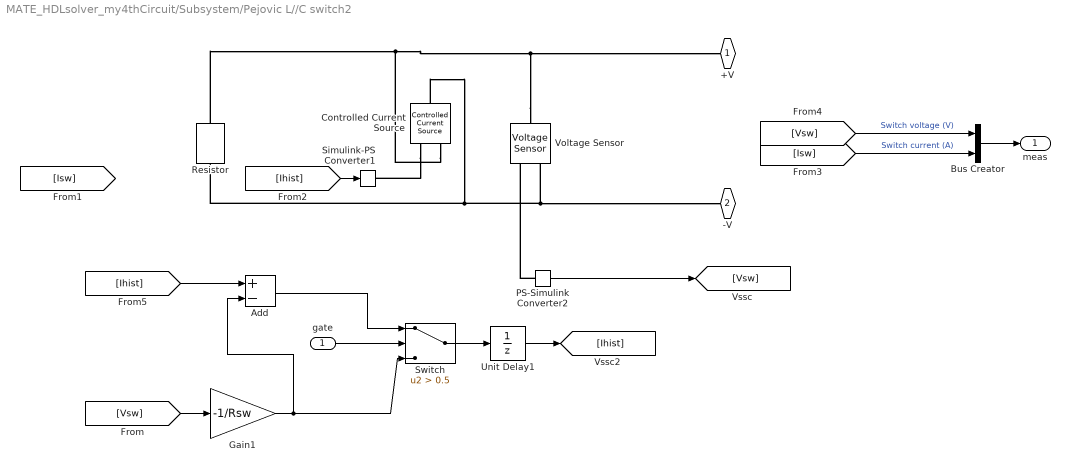
== system MATE_HDLsolver_my4thCircuit/Subsystem/Pejovic L//C switch2 ==
  gate : Inport
  Add : Sum  Inputs=+-
  Bus Creator : BusCreator  Inputs=2
  Controlled Current Source : fl_lib/Electrical/Electrical Sources/Controlled Current Source
  Gain1 : Gain  Gain=-1/Rsw
  PS-Simulink Converter2 : nesl_utility/PS-Simulink Converter  PhysicalDomain=network_engine_domain  SubClassName=ps_output  LeftPortType=input  RightPortType=output  PseudoPeriodic=off  Frequencies=[]  VectorFormat=inherit  Unit=inherit  AffineConversion=off
  Resistor : fl_lib/Electrical/Electrical Elements/Resistor  R=Rsw Ohm  i_specify=off  i_priority=None  i=0 A  i_nominal_specify=off  i_nominal_value=1  i_nominal_unit=A  v_specify=off  v_priority=None  v=0 V  v_nominal_specify=off  v_nominal_value=1  v_nominal_unit=V
  Simulink-PS Converter1 : nesl_utility/Simulink-PS Converter  PhysicalDomain=network_engine_domain  SubClassName=ps_input  LeftPortType=input  RightPortType=output  PseudoPeriodic=off  Frequencies=[]  NoiseDistribution=none  NoiseParameters=[]  Unit=1  AffineConversion=off  FilteringAndDerivatives=provide  SimscapeFilterOrder=1  InputFilterTimeConstant=0.001  UdotUserProvided=0
  Switch : Switch  Criteria=u2 > Threshold  Threshold=0.5  SaturateOnIntegerOverflow=off  InputSameDT=off
  Unit Delay1 : UnitDelay  SampleTime=-1  HasFrameUpgradeWarning=on
  Voltage Sensor : fl_lib/Electrical/Electrical Sensors/Voltage Sensor
  +V : PMIOPort  Side=Left
  -V : PMIOPort  Port=2  Side=Right
  meas : Outport
  wires:
  Unit Delay1/1 -> [Ihist]
  Add/1 -> Switch/1
  Gain1/1 -> Add/2, Switch/3
  [Ihist] -> Add/1
  PS-Simulink Converter2/1 -> [Vsw]
  gate/1 -> Switch/2
  [Vsw] -> Gain1/1
  Switch/1 -> Unit Delay1/1
  [Ihist] -> Simulink-PS Converter1/1
  [Isw] -> Bus Creator/2  "Switch current (A)"
  [Vsw] -> Bus Creator/1  "Switch voltage (V)"
  Bus Creator/1 -> meas/1
  connections:
  Resistor/RConn1 -- Controlled Current Source/LConn1 -- Voltage Sensor/RConn2 -- -V/RConn1
  PS-Simulink Converter2/LConn1 -- Voltage Sensor/RConn1
  Controlled Current Source/RConn1 -- Simulink-PS Converter1/RConn1
  Voltage Sensor/LConn1 -- +V/RConn1 -- Controlled Current Source/RConn2 -- Resistor/LConn1

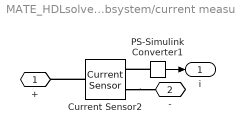
== system MATE_HDLsolver_my4thCircuit/Subsystem/current measure ==
  Current Sensor2 : fl_lib/Electrical/Electrical Sensors/Current Sensor
  PS-Simulink Converter1 : nesl_utility/PS-Simulink Converter  PhysicalDomain=network_engine_domain  SubClassName=ps_output  LeftPortType=input  RightPortType=output  PseudoPeriodic=off  Frequencies=[]  VectorFormat=inherit  Unit=inherit  AffineConversion=off
  + : PMIOPort  Side=Left
  - : PMIOPort  Port=2  Side=Right
  i : Outport
  wires:
  PS-Simulink Converter1/1 -> i/1
  connections:
  PS-Simulink Converter1/LConn1 -- Current Sensor2/RConn1
  Current Sensor2/LConn1 -- +/RConn1
  Current Sensor2/RConn2 -- -/RConn1
